simulink library "AFCToolbox2023a"  (R2023a)
settings: Solver=VariableStepAuto  StartTime=0.0  StopTime=10.0  RelTol=1e-3
undefined symbols (not defined in the file or in its folder): AFC5Toolbox_SimuMoudle, AFCToolbox, ax, ay, az, btnSample, C_d, C_dm, C_m, C_t, Control, d, declination_table, dp0, dp1, dp2, dp3, dt, euler_0, g0, I_xyz, inclination_table, J_m, lmd_high, lmd_low, lp_acc_knoise, lp_acc_max, lp_acc_min, lp_acc_seed, lp_GPS_BL_max, lp_GPS_BL_min, lp_GPS_H_max, lp_GPS_H_min, lp_GPS_knoise, lp_GPS_seed, lp_GPS_vel_max, lp_GPS_vel_min, lp_gyro_knoise, lp_gyro_max, lp_gyro_min, lp_gyro_seed, lp_hf_vwind, lp_hs_vwind_interp, lp_kaerorho, lp_kaeroT, lp_kIxyz, lp_kmass, lp_momentx_A0, lp_momentx_Af, lp_momentx_ts, lp_momenty_A0, lp_momenty_Af, lp_momenty_ts, lp_momentz_A0, lp_momentz_Af, lp_momentz_ts, lp_vf_vwind, lp_vs_vwind_interp, lp_vwind_thetax, lp_vwind_thetaz ... (+54)
libraries: $bdroot x104, simulink x75, etargetslib x32, sharedtransform x13, simulink_extras x12, dspstat3 x11, aerolibconvert2 x9, aerolibtransform2 x3, aerolibutil x2, matrix_library x1
(part 9 of 10)

== matlab function AFCToolbox2023a/基础导航算法模型库/ECL EKF/Subsystem/Subsystem2/Predict Covariance ==
  data: delta_ang input; delta_vel input; P output; states input; P input single; dt input; accel_bias_inhibit input
function P  = PredictCovariance(delta_ang, ...%imu_sample_delayed.delta_ang
    delta_vel,...%imu_sample_delayed.delta_vel
    states,...% previous state vector (4x1 quaternion, 3x1 velocity, 3x1 position, 3x1 delAng bias, 3x1 delVel bias)
    P, dt, ... % IMU and prediction time step
    accel_bias_inhibit)% inhibited for the specified axis
    

%  the current status of the filter control modes
%% control status flags
control_status_flags.wind  = 1;
control_status_flags.mag_3D = 1;

% tuning parameters
%% InitCovariance params
params.gps_vel_noise = 0.5;
params.gps_pos_noise = 0.5;
params.pos_noaid_noise = 10;
params.baro_noise = 2;
params.switch_on_gyro_bias = 0.1;
params.switch_on_accel_bias = 0.2;
params.mag_noise = 0.05;
params.initial_wind_uncertainty = 1;
params.gyro_noise = 0.00001;
params.accel_noise = 0.35;
%% PredictCovariance params
params.gyro_bias_p_noise = 0.0001;
params.accel_bias_p_noise = 0.001;
params.mage_p_noise = 0.001;
params.magb_p_noise = 0.0001;
params.wind_vel_p_noise = 0.5;


%% assign intermediate state variables
% quaternion
states_quat_nominal = normQuat(states(1:4));
q0 = states_quat_nominal(1);
q1 = states_quat_nominal(2);
q2 = states_quat_nominal(3);
q3 = states_quat_nominal(4);
% delta angle 
dax = delta_ang(1);
day = delta_ang(2);
daz = delta_ang(3);
% delta velocity
dvx = delta_vel(1);
dvy = delta_vel(2);
dvz = delta_vel(3);
% delta angle bias
dax_b = states(11);
day_b = states(12);
daz_b = states(13);
% delta velocity bias
dvx_b = states(14);
dvy_b = states(15);
dvz_b = states(16);

% convert rate of change of rate gyro bias (rad/s**2) as specified by the parameter to an expected change in delta angle (rad) since the last update
d_ang_bias_sig = dt * dt * params.gyro_bias_p_noise;

% convert rate of change of accelerometer bias (m/s**3) as specified by the parameter to an expected change in delta velocity (m/s) since the last update
d_vel_bias_sig = dt * dt * params.accel_bias_p_noise;

%% This process noise determines the rate of estimation of IMU bias errors
% Set filter state process noise other than IMU errors, which are already
% built into the derived covariance prediction equations.
mag_I_sig = dt * params.mage_p_noise;
mag_B_sig = dt * params.magb_p_noise;
wind_vel_sig = dt * params.wind_vel_p_noise;
process_noise = [zeros(1,10), d_ang_bias_sig*[1 1 1], d_vel_bias_sig*[1 1 1], mag_I_sig*[1 1 1], mag_B_sig*[1 1 1], wind_vel_sig*[1 1]].^2;

%% assign IMU noise variances
% Specify the noise variance on the IMU delta angles and delta velocities
daxVar = (dt * params.gyro_noise)^2;
dayVar = daxVar;
dazVar = daxVar;
dvxVar = (dt * params.accel_noise)^2;
dvyVar = dvxVar;
dvzVar = dvxVar;

%% intermediate calculations——求解223条赋值语句，得出中间变量
PS0 = power(q1, 2);
PS1 = 0.25*daxVar;
PS2 = power(q2, 2);
PS3 = 0.25*dayVar;
PS4 = power(q3, 2);
PS5 = 0.25*dazVar;
PS6 = 0.5*q1;
PS7 = 0.5*q2;
PS8 = C_P(P,10,11)*PS7;
PS9 = 0.5*q3;
PS10 = C_P(P,10,12)*PS9;
PS11 = 0.5*dax - 0.5*dax_b;
PS12 = 0.5*day - 0.5*day_b;
PS13 = 0.5*daz - 0.5*daz_b;
PS14 = C_P(P,0,10) - C_P(P,1,10)*PS11 + C_P(P,10,10)*PS6 - C_P(P,2,10)*PS12 - C_P(P,3,10)*PS13 + PS10 + PS8;
PS15 = C_P(P,10,11)*PS6;
PS16 = C_P(P,11,12)*PS9;
PS17 = C_P(P,0,11) - C_P(P,1,11)*PS11 + C_P(P,11,11)*PS7 - C_P(P,2,11)*PS12 - C_P(P,3,11)*PS13 + PS15 + PS16;
PS18 = C_P(P,10,12)*PS6;
PS19 = C_P(P,11,12)*PS7;
PS20 = C_P(P,0,12) - C_P(P,1,12)*PS11 + C_P(P,12,12)*PS9 - C_P(P,2,12)*PS12 - C_P(P,3,12)*PS13 + PS18 + PS19;
PS21 = C_P(P,1,2)*PS12;
PS22 = -C_P(P,1,3)*PS13;
PS23 = C_P(P,0,1) - C_P(P,1,1)*PS11 + C_P(P,1,10)*PS6 + C_P(P,1,11)*PS7 + C_P(P,1,12)*PS9 - PS21 + PS22;
PS24 = -C_P(P,1,2)*PS11;
PS25 = C_P(P,2,3)*PS13;
PS26 = C_P(P,0,2) + C_P(P,2,10)*PS6 + C_P(P,2,11)*PS7 + C_P(P,2,12)*PS9 - C_P(P,2,2)*PS12 + PS24 - PS25;
PS27 = C_P(P,1,3)*PS11;
PS28 = -C_P(P,2,3)*PS12;
PS29 = C_P(P,0,3) + C_P(P,3,10)*PS6 + C_P(P,3,11)*PS7 + C_P(P,3,12)*PS9 - C_P(P,3,3)*PS13 - PS27 + PS28;
PS30 = C_P(P,0,1)*PS11;
PS31 = C_P(P,0,2)*PS12;
PS32 = C_P(P,0,3)*PS13;
PS33 = C_P(P,0,0) + C_P(P,0,10)*PS6 + C_P(P,0,11)*PS7 + C_P(P,0,12)*PS9 - PS30 - PS31 - PS32;
PS34 = 0.5*q0;
PS35 = q2*q3;
PS36 = q0*q1;
PS37 = q1*q3;
PS38 = q0*q2;
PS39 = q1*q2;
PS40 = q0*q3;
PS41 = 2*PS2;
PS42 = 2*PS4 - 1;
PS43 = PS41 + PS42;
PS44 = C_P(P,0,13) - C_P(P,1,13)*PS11 + C_P(P,10,13)*PS6 + C_P(P,11,13)*PS7 + C_P(P,12,13)*PS9 - C_P(P,2,13)*PS12 - C_P(P,3,13)*PS13;
PS45 = PS37 + PS38;
PS46 = C_P(P,0,15) - C_P(P,1,15)*PS11 + C_P(P,10,15)*PS6 + C_P(P,11,15)*PS7 + C_P(P,12,15)*PS9 - C_P(P,2,15)*PS12 - C_P(P,3,15)*PS13;
PS47 = 2*PS46;
PS48 = dvy - dvy_b;
PS49 = PS48*q0;
PS50 = dvz - dvz_b;
PS51 = PS50*q1;
PS52 = dvx - dvx_b;
PS53 = PS52*q3;
PS54 = PS49 - PS51 + 2*PS53;
PS55 = 2*PS29;
PS56 = -PS39 + PS40;
PS57 = C_P(P,0,14) - C_P(P,1,14)*PS11 + C_P(P,10,14)*PS6 + C_P(P,11,14)*PS7 + C_P(P,12,14)*PS9 - C_P(P,2,14)*PS12 - C_P(P,3,14)*PS13;
PS58 = 2*PS57;
PS59 = PS48*q2;
PS60 = PS50*q3;
PS61 = PS59 + PS60;
PS62 = 2*PS23;
PS63 = PS50*q2;
PS64 = PS48*q3;
PS65 = -PS64;
PS66 = PS63 + PS65;
PS67 = 2*PS33;
PS68 = PS50*q0;
PS69 = PS48*q1;
PS70 = PS52*q2;
PS71 = PS68 + PS69 - 2*PS70;
PS72 = 2*PS26;
PS73 = C_P(P,0,4) - C_P(P,1,4)*PS11 - C_P(P,2,4)*PS12 - C_P(P,3,4)*PS13 + C_P(P,4,10)*PS6 + C_P(P,4,11)*PS7 + C_P(P,4,12)*PS9;
PS74 = 2*PS0;
PS75 = PS42 + PS74;
PS76 = PS39 + PS40;
PS77 = 2*PS44;
PS78 = PS51 - PS53;
PS79 = -PS70;
PS80 = PS68 + 2*PS69 + PS79;
PS81 = -PS35 + PS36;
PS82 = PS52*q1;
PS83 = PS60 + PS82;
PS84 = PS52*q0;
PS85 = PS63 - 2*PS64 + PS84;
PS86 = C_P(P,0,5) - C_P(P,1,5)*PS11 - C_P(P,2,5)*PS12 - C_P(P,3,5)*PS13 + C_P(P,5,10)*PS6 + C_P(P,5,11)*PS7 + C_P(P,5,12)*PS9;
PS87 = PS41 + PS74 - 1;
PS88 = PS35 + PS36;
PS89 = 2*PS63 + PS65 + PS84;
PS90 = -PS37 + PS38;
PS91 = PS59 + PS82;
PS92 = PS69 + PS79;
PS93 = PS49 - 2*PS51 + PS53;
PS94 = C_P(P,0,6) - C_P(P,1,6)*PS11 - C_P(P,2,6)*PS12 - C_P(P,3,6)*PS13 + C_P(P,6,10)*PS6 + C_P(P,6,11)*PS7 + C_P(P,6,12)*PS9;
PS95 = power(q0, 2);
PS96 = -C_P(P,10,11)*PS34;
PS97 = C_P(P,0,11)*PS11 + C_P(P,1,11) + C_P(P,11,11)*PS9 + C_P(P,2,11)*PS13 - C_P(P,3,11)*PS12 - PS19 + PS96;
PS98 = C_P(P,0,2)*PS13;
PS99 = C_P(P,0,3)*PS12;
PS100 = C_P(P,0,0)*PS11 + C_P(P,0,1) - C_P(P,0,10)*PS34 + C_P(P,0,11)*PS9 - C_P(P,0,12)*PS7 + PS98 - PS99;
PS101 = C_P(P,0,2)*PS11;
PS102 = C_P(P,1,2) - C_P(P,2,10)*PS34 + C_P(P,2,11)*PS9 - C_P(P,2,12)*PS7 + C_P(P,2,2)*PS13 + PS101 + PS28;
PS103 = C_P(P,10,11)*PS9;
PS104 = C_P(P,10,12)*PS7;
PS105 = C_P(P,0,10)*PS11 + C_P(P,1,10) - C_P(P,10,10)*PS34 + C_P(P,2,10)*PS13 - C_P(P,3,10)*PS12 + PS103 - PS104;
PS106 = -C_P(P,10,12)*PS34;
PS107 = C_P(P,0,12)*PS11 + C_P(P,1,12) - C_P(P,12,12)*PS7 + C_P(P,2,12)*PS13 - C_P(P,3,12)*PS12 + PS106 + PS16;
PS108 = C_P(P,0,3)*PS11;
PS109 = C_P(P,1,3) - C_P(P,3,10)*PS34 + C_P(P,3,11)*PS9 - C_P(P,3,12)*PS7 - C_P(P,3,3)*PS12 + PS108 + PS25;
PS110 = C_P(P,1,2)*PS13;
PS111 = C_P(P,1,3)*PS12;
PS112 = C_P(P,1,1) - C_P(P,1,10)*PS34 + C_P(P,1,11)*PS9 - C_P(P,1,12)*PS7 + PS110 - PS111 + PS30;
PS113 = C_P(P,0,13)*PS11 + C_P(P,1,13) - C_P(P,10,13)*PS34 + C_P(P,11,13)*PS9 - C_P(P,12,13)*PS7 + C_P(P,2,13)*PS13 - C_P(P,3,13)*PS12;
PS114 = C_P(P,0,15)*PS11 + C_P(P,1,15) - C_P(P,10,15)*PS34 + C_P(P,11,15)*PS9 - C_P(P,12,15)*PS7 + C_P(P,2,15)*PS13 - C_P(P,3,15)*PS12;
PS115 = 2*PS114;
PS116 = 2*PS109;
PS117 = C_P(P,0,14)*PS11 + C_P(P,1,14) - C_P(P,10,14)*PS34 + C_P(P,11,14)*PS9 - C_P(P,12,14)*PS7 + C_P(P,2,14)*PS13 - C_P(P,3,14)*PS12;
PS118 = 2*PS117;
PS119 = 2*PS112;
PS120 = 2*PS100;
PS121 = 2*PS102;
PS122 = C_P(P,0,4)*PS11 + C_P(P,1,4) + C_P(P,2,4)*PS13 - C_P(P,3,4)*PS12 - C_P(P,4,10)*PS34 + C_P(P,4,11)*PS9 - C_P(P,4,12)*PS7;
PS123 = 2*PS113;
PS124 = C_P(P,0,5)*PS11 + C_P(P,1,5) + C_P(P,2,5)*PS13 - C_P(P,3,5)*PS12 - C_P(P,5,10)*PS34 + C_P(P,5,11)*PS9 - C_P(P,5,12)*PS7;
PS125 = C_P(P,0,6)*PS11 + C_P(P,1,6) + C_P(P,2,6)*PS13 - C_P(P,3,6)*PS12 - C_P(P,6,10)*PS34 + C_P(P,6,11)*PS9 - C_P(P,6,12)*PS7;
PS126 = -C_P(P,11,12)*PS34;
PS127 = C_P(P,0,12)*PS12 - C_P(P,1,12)*PS13 + C_P(P,12,12)*PS6 + C_P(P,2,12) + C_P(P,3,12)*PS11 - PS10 + PS126;
PS128 = C_P(P,2,3) - C_P(P,3,10)*PS9 - C_P(P,3,11)*PS34 + C_P(P,3,12)*PS6 + C_P(P,3,3)*PS11 + PS22 + PS99;
PS129 = C_P(P,0,1)*PS13;
PS130 = C_P(P,0,0)*PS12 - C_P(P,0,10)*PS9 - C_P(P,0,11)*PS34 + C_P(P,0,12)*PS6 + C_P(P,0,2) + PS108 - PS129;
PS131 = C_P(P,11,12)*PS6;
PS132 = C_P(P,0,11)*PS12 - C_P(P,1,11)*PS13 - C_P(P,11,11)*PS34 + C_P(P,2,11) + C_P(P,3,11)*PS11 - PS103 + PS131;
PS133 = C_P(P,0,10)*PS12 - C_P(P,1,10)*PS13 - C_P(P,10,10)*PS9 + C_P(P,2,10) + C_P(P,3,10)*PS11 + PS18 + PS96;
PS134 = C_P(P,0,1)*PS12;
PS135 = -C_P(P,1,1)*PS13 - C_P(P,1,10)*PS9 - C_P(P,1,11)*PS34 + C_P(P,1,12)*PS6 + C_P(P,1,2) + PS134 + PS27;
PS136 = C_P(P,2,3)*PS11;
PS137 = -C_P(P,2,10)*PS9 - C_P(P,2,11)*PS34 + C_P(P,2,12)*PS6 + C_P(P,2,2) - PS110 + PS136 + PS31;
PS138 = C_P(P,0,13)*PS12 - C_P(P,1,13)*PS13 - C_P(P,10,13)*PS9 - C_P(P,11,13)*PS34 + C_P(P,12,13)*PS6 + C_P(P,2,13) + C_P(P,3,13)*PS11;
PS139 = C_P(P,0,15)*PS12 - C_P(P,1,15)*PS13 - C_P(P,10,15)*PS9 - C_P(P,11,15)*PS34 + C_P(P,12,15)*PS6 + C_P(P,2,15) + C_P(P,3,15)*PS11;
PS140 = 2*PS139;
PS141 = 2*PS128;
PS142 = C_P(P,0,14)*PS12 - C_P(P,1,14)*PS13 - C_P(P,10,14)*PS9 - C_P(P,11,14)*PS34 + C_P(P,12,14)*PS6 + C_P(P,2,14) + C_P(P,3,14)*PS11;
PS143 = 2*PS142;
PS144 = 2*PS135;
PS145 = 2*PS130;
PS146 = 2*PS137;
PS147 = C_P(P,0,4)*PS12 - C_P(P,1,4)*PS13 + C_P(P,2,4) + C_P(P,3,4)*PS11 - C_P(P,4,10)*PS9 - C_P(P,4,11)*PS34 + C_P(P,4,12)*PS6;
PS148 = 2*PS138;
PS149 = C_P(P,0,5)*PS12 - C_P(P,1,5)*PS13 + C_P(P,2,5) + C_P(P,3,5)*PS11 - C_P(P,5,10)*PS9 - C_P(P,5,11)*PS34 + C_P(P,5,12)*PS6;
PS150 = C_P(P,0,6)*PS12 - C_P(P,1,6)*PS13 + C_P(P,2,6) + C_P(P,3,6)*PS11 - C_P(P,6,10)*PS9 - C_P(P,6,11)*PS34 + C_P(P,6,12)*PS6;
PS151 = C_P(P,0,10)*PS13 + C_P(P,1,10)*PS12 + C_P(P,10,10)*PS7 - C_P(P,2,10)*PS11 + C_P(P,3,10) + PS106 - PS15;
PS152 = C_P(P,1,1)*PS12 + C_P(P,1,10)*PS7 - C_P(P,1,11)*PS6 - C_P(P,1,12)*PS34 + C_P(P,1,3) + PS129 + PS24;
PS153 = C_P(P,0,0)*PS13 + C_P(P,0,10)*PS7 - C_P(P,0,11)*PS6 - C_P(P,0,12)*PS34 + C_P(P,0,3) - PS101 + PS134;
PS154 = C_P(P,0,12)*PS13 + C_P(P,1,12)*PS12 - C_P(P,12,12)*PS34 - C_P(P,2,12)*PS11 + C_P(P,3,12) + PS104 - PS131;
PS155 = C_P(P,0,11)*PS13 + C_P(P,1,11)*PS12 - C_P(P,11,11)*PS6 - C_P(P,2,11)*PS11 + C_P(P,3,11) + PS126 + PS8;
PS156 = C_P(P,2,10)*PS7 - C_P(P,2,11)*PS6 - C_P(P,2,12)*PS34 - C_P(P,2,2)*PS11 + C_P(P,2,3) + PS21 + PS98;
PS157 = C_P(P,3,10)*PS7 - C_P(P,3,11)*PS6 - C_P(P,3,12)*PS34 + C_P(P,3,3) + PS111 - PS136 + PS32;
PS158 = C_P(P,0,13)*PS13 + C_P(P,1,13)*PS12 + C_P(P,10,13)*PS7 - C_P(P,11,13)*PS6 - C_P(P,12,13)*PS34 - C_P(P,2,13)*PS11 + C_P(P,3,13);
PS159 = C_P(P,0,15)*PS13 + C_P(P,1,15)*PS12 + C_P(P,10,15)*PS7 - C_P(P,11,15)*PS6 - C_P(P,12,15)*PS34 - C_P(P,2,15)*PS11 + C_P(P,3,15);
PS160 = 2*PS159;
PS161 = 2*PS157;
PS162 = C_P(P,0,14)*PS13 + C_P(P,1,14)*PS12 + C_P(P,10,14)*PS7 - C_P(P,11,14)*PS6 - C_P(P,12,14)*PS34 - C_P(P,2,14)*PS11 + C_P(P,3,14);
PS163 = 2*PS162;
PS164 = 2*PS152;
PS165 = 2*PS153;
PS166 = 2*PS156;
PS167 = C_P(P,0,4)*PS13 + C_P(P,1,4)*PS12 - C_P(P,2,4)*PS11 + C_P(P,3,4) + C_P(P,4,10)*PS7 - C_P(P,4,11)*PS6 - C_P(P,4,12)*PS34;
PS168 = 2*PS158;
PS169 = C_P(P,0,5)*PS13 + C_P(P,1,5)*PS12 - C_P(P,2,5)*PS11 + C_P(P,3,5) + C_P(P,5,10)*PS7 - C_P(P,5,11)*PS6 - C_P(P,5,12)*PS34;
PS170 = C_P(P,0,6)*PS13 + C_P(P,1,6)*PS12 - C_P(P,2,6)*PS11 + C_P(P,3,6) + C_P(P,6,10)*PS7 - C_P(P,6,11)*PS6 - C_P(P,6,12)*PS34;
PS171 = 2*PS45;
PS172 = 2*PS56;
PS173 = 2*PS61;
PS174 = 2*PS66;
PS175 = 2*PS71;
PS176 = 2*PS54;
PS177 = C_P(P,0,13)*PS174 + C_P(P,1,13)*PS173 + C_P(P,13,13)*PS43 + C_P(P,13,14)*PS172 - C_P(P,13,15)*PS171 + C_P(P,2,13)*PS175 - C_P(P,3,13)*PS176 + C_P(P,4,13);
PS178 = C_P(P,0,15)*PS174 + C_P(P,1,15)*PS173 + C_P(P,13,15)*PS43 + C_P(P,14,15)*PS172 - C_P(P,15,15)*PS171 + C_P(P,2,15)*PS175 - C_P(P,3,15)*PS176 + C_P(P,4,15);
PS179 = C_P(P,0,3)*PS174 + C_P(P,1,3)*PS173 + C_P(P,2,3)*PS175 + C_P(P,3,13)*PS43 + C_P(P,3,14)*PS172 - C_P(P,3,15)*PS171 - C_P(P,3,3)*PS176 + C_P(P,3,4);
PS180 = C_P(P,0,14)*PS174 + C_P(P,1,14)*PS173 + C_P(P,13,14)*PS43 + C_P(P,14,14)*PS172 - C_P(P,14,15)*PS171 + C_P(P,2,14)*PS175 - C_P(P,3,14)*PS176 + C_P(P,4,14);
PS181 = C_P(P,0,1)*PS174 + C_P(P,1,1)*PS173 + C_P(P,1,13)*PS43 + C_P(P,1,14)*PS172 - C_P(P,1,15)*PS171 + C_P(P,1,2)*PS175 - C_P(P,1,3)*PS176 + C_P(P,1,4);
PS182 = C_P(P,0,0)*PS174 + C_P(P,0,1)*PS173 + C_P(P,0,13)*PS43 + C_P(P,0,14)*PS172 - C_P(P,0,15)*PS171 + C_P(P,0,2)*PS175 - C_P(P,0,3)*PS176 + C_P(P,0,4);
PS183 = C_P(P,0,2)*PS174 + C_P(P,1,2)*PS173 + C_P(P,2,13)*PS43 + C_P(P,2,14)*PS172 - C_P(P,2,15)*PS171 + C_P(P,2,2)*PS175 - C_P(P,2,3)*PS176 + C_P(P,2,4);
PS184 = 4*dvyVar;
PS185 = 4*dvzVar;
PS186 = C_P(P,0,4)*PS174 + C_P(P,1,4)*PS173 + C_P(P,2,4)*PS175 - C_P(P,3,4)*PS176 + C_P(P,4,13)*PS43 + C_P(P,4,14)*PS172 - C_P(P,4,15)*PS171 + C_P(P,4,4);
PS187 = 2*PS177;
PS188 = 2*PS182;
PS189 = 2*PS181;
PS190 = 2*PS81;
PS191 = 2*PS183;
PS192 = 2*PS179;
PS193 = 2*PS76;
PS194 = PS43*dvxVar;
PS195 = PS75*dvyVar;
PS196 = C_P(P,0,5)*PS174 + C_P(P,1,5)*PS173 + C_P(P,2,5)*PS175 - C_P(P,3,5)*PS176 + C_P(P,4,5) + C_P(P,5,13)*PS43 + C_P(P,5,14)*PS172 - C_P(P,5,15)*PS171;
PS197 = 2*PS88;
PS198 = PS87*dvzVar;
PS199 = 2*PS90;
PS200 = C_P(P,0,6)*PS174 + C_P(P,1,6)*PS173 + C_P(P,2,6)*PS175 - C_P(P,3,6)*PS176 + C_P(P,4,6) + C_P(P,6,13)*PS43 + C_P(P,6,14)*PS172 - C_P(P,6,15)*PS171;
PS201 = 2*PS83;
PS202 = 2*PS78;
PS203 = 2*PS85;
PS204 = 2*PS80;
PS205 = -C_P(P,0,14)*PS202 - C_P(P,1,14)*PS204 - C_P(P,13,14)*PS193 + C_P(P,14,14)*PS75 + C_P(P,14,15)*PS190 + C_P(P,2,14)*PS201 + C_P(P,3,14)*PS203 + C_P(P,5,14);
PS206 = -C_P(P,0,13)*PS202 - C_P(P,1,13)*PS204 - C_P(P,13,13)*PS193 + C_P(P,13,14)*PS75 + C_P(P,13,15)*PS190 + C_P(P,2,13)*PS201 + C_P(P,3,13)*PS203 + C_P(P,5,13);
PS207 = -C_P(P,0,0)*PS202 - C_P(P,0,1)*PS204 - C_P(P,0,13)*PS193 + C_P(P,0,14)*PS75 + C_P(P,0,15)*PS190 + C_P(P,0,2)*PS201 + C_P(P,0,3)*PS203 + C_P(P,0,5);
PS208 = -C_P(P,0,1)*PS202 - C_P(P,1,1)*PS204 - C_P(P,1,13)*PS193 + C_P(P,1,14)*PS75 + C_P(P,1,15)*PS190 + C_P(P,1,2)*PS201 + C_P(P,1,3)*PS203 + C_P(P,1,5);
PS209 = -C_P(P,0,15)*PS202 - C_P(P,1,15)*PS204 - C_P(P,13,15)*PS193 + C_P(P,14,15)*PS75 + C_P(P,15,15)*PS190 + C_P(P,2,15)*PS201 + C_P(P,3,15)*PS203 + C_P(P,5,15);
PS210 = -C_P(P,0,2)*PS202 - C_P(P,1,2)*PS204 - C_P(P,2,13)*PS193 + C_P(P,2,14)*PS75 + C_P(P,2,15)*PS190 + C_P(P,2,2)*PS201 + C_P(P,2,3)*PS203 + C_P(P,2,5);
PS211 = -C_P(P,0,3)*PS202 - C_P(P,1,3)*PS204 + C_P(P,2,3)*PS201 - C_P(P,3,13)*PS193 + C_P(P,3,14)*PS75 + C_P(P,3,15)*PS190 + C_P(P,3,3)*PS203 + C_P(P,3,5);
PS212 = 4*dvxVar;
PS213 = -C_P(P,0,5)*PS202 - C_P(P,1,5)*PS204 + C_P(P,2,5)*PS201 + C_P(P,3,5)*PS203 - C_P(P,5,13)*PS193 + C_P(P,5,14)*PS75 + C_P(P,5,15)*PS190 + C_P(P,5,5);
PS214 = 2*PS89;
PS215 = 2*PS91;
PS216 = 2*PS92;
PS217 = 2*PS93;
PS218 = -C_P(P,0,6)*PS202 - C_P(P,1,6)*PS204 + C_P(P,2,6)*PS201 + C_P(P,3,6)*PS203 + C_P(P,5,6) - C_P(P,6,13)*PS193 + C_P(P,6,14)*PS75 + C_P(P,6,15)*PS190;
PS219 = C_P(P,0,15)*PS216 + C_P(P,1,15)*PS217 + C_P(P,13,15)*PS199 - C_P(P,14,15)*PS197 + C_P(P,15,15)*PS87 - C_P(P,2,15)*PS214 + C_P(P,3,15)*PS215 + C_P(P,6,15);
PS220 = C_P(P,0,14)*PS216 + C_P(P,1,14)*PS217 + C_P(P,13,14)*PS199 - C_P(P,14,14)*PS197 + C_P(P,14,15)*PS87 - C_P(P,2,14)*PS214 + C_P(P,3,14)*PS215 + C_P(P,6,14);
PS221 = C_P(P,0,13)*PS216 + C_P(P,1,13)*PS217 + C_P(P,13,13)*PS199 - C_P(P,13,14)*PS197 + C_P(P,13,15)*PS87 - C_P(P,2,13)*PS214 + C_P(P,3,13)*PS215 + C_P(P,6,13);
PS222 = C_P(P,0,6)*PS216 + C_P(P,1,6)*PS217 - C_P(P,2,6)*PS214 + C_P(P,3,6)*PS215 + C_P(P,6,13)*PS199 - C_P(P,6,14)*PS197 + C_P(P,6,15)*PS87 + C_P(P,6,6);

%% caculate covariances
% initialize covariances
nextP_ = zeros(24,24);
% calculate variances and upper diagonal covariances for QUATERNION, VELOCITY, POSITION AND GYRO BIAS states
nextP_(1,1) = PS0*PS1 - PS11*PS23 - PS12*PS26 - PS13*PS29 + PS14*PS6 + PS17*PS7 + PS2*PS3 + PS20*PS9 + PS33 + PS4*PS5;
nextP_(1,2) = -PS1*PS36 + PS11*PS33 - PS12*PS29 + PS13*PS26 - PS14*PS34 + PS17*PS9 - PS20*PS7 + PS23 + PS3*PS35 - PS35*PS5;
nextP_(2,2) = PS1*PS95 + PS100*PS11 + PS102*PS13 - PS105*PS34 - PS107*PS7 - PS109*PS12 + PS112 + PS2*PS5 + PS3*PS4 + PS9*PS97;

nextP_(1,3) = -PS1*PS37 + PS11*PS29 + PS12*PS33 - PS13*PS23 - PS14*PS9 - PS17*PS34 + PS20*PS6 + PS26 - PS3*PS38 + PS37*PS5;
nextP_(2,3) = PS1*PS40 + PS100*PS12 + PS102 - PS105*PS9 + PS107*PS6 + PS109*PS11 - PS112*PS13 - PS3*PS40 - PS34*PS97 - PS39*PS5;
nextP_(3,3) = PS0*PS5 + PS1*PS4 + PS11*PS128 + PS12*PS130 + PS127*PS6 - PS13*PS135 - PS132*PS34 - PS133*PS9 + PS137 + PS3*PS95;

nextP_(1,4) = PS1*PS39 - PS11*PS26 + PS12*PS23 + PS13*PS33 + PS14*PS7 - PS17*PS6 - PS20*PS34 + PS29 - PS3*PS39 - PS40*PS5;
nextP_(2,4) = -PS1*PS38 + PS100*PS13 - PS102*PS11 + PS105*PS7 - PS107*PS34 + PS109 + PS112*PS12 - PS3*PS37 + PS38*PS5 - PS6*PS97;
nextP_(3,4) = -PS1*PS35 - PS11*PS137 + PS12*PS135 - PS127*PS34 + PS128 + PS13*PS130 - PS132*PS6 + PS133*PS7 + PS3*PS36 - PS36*PS5;
nextP_(4,4) = PS0*PS3 + PS1*PS2 - PS11*PS156 + PS12*PS152 + PS13*PS153 + PS151*PS7 - PS154*PS34 - PS155*PS6 + PS157 + PS5*PS95;

nextP_(1,5) = PS43*PS44 - PS45*PS47 - PS54*PS55 + PS56*PS58 + PS61*PS62 + PS66*PS67 + PS71*PS72 + PS73;
nextP_(2,5) = PS113*PS43 - PS115*PS45 - PS116*PS54 + PS118*PS56 + PS119*PS61 + PS120*PS66 + PS121*PS71 + PS122;
nextP_(3,5) = PS138*PS43 - PS140*PS45 - PS141*PS54 + PS143*PS56 + PS144*PS61 + PS145*PS66 + PS146*PS71 + PS147;
nextP_(4,5) = PS158*PS43 - PS160*PS45 - PS161*PS54 + PS163*PS56 + PS164*PS61 + PS165*PS66 + PS166*PS71 + PS167;
nextP_(5,5) = -PS171*PS178 + PS172*PS180 + PS173*PS181 + PS174*PS182 + PS175*PS183 - PS176*PS179 + PS177*PS43 + PS184*power(PS56, 2) + PS185*power(PS45, 2) + PS186 + power(PS43, 2)*dvxVar;

nextP_(1,6) = PS47*PS81 + PS55*PS85 + PS57*PS75 - PS62*PS80 - PS67*PS78 + PS72*PS83 - PS76*PS77 + PS86;
nextP_(2,6) = PS115*PS81 + PS116*PS85 + PS117*PS75 - PS119*PS80 - PS120*PS78 + PS121*PS83 - PS123*PS76 + PS124;
nextP_(3,6) = PS140*PS81 + PS141*PS85 + PS142*PS75 - PS144*PS80 - PS145*PS78 + PS146*PS83 - PS148*PS76 + PS149;
nextP_(4,6) = PS160*PS81 + PS161*PS85 + PS162*PS75 - PS164*PS80 - PS165*PS78 + PS166*PS83 - PS168*PS76 + PS169;
nextP_(5,6) = PS172*PS195 + PS178*PS190 + PS180*PS75 - PS185*PS45*PS81 - PS187*PS76 - PS188*PS78 - PS189*PS80 + PS191*PS83 + PS192*PS85 - PS193*PS194 + PS196;
nextP_(6,6) = PS185*power(PS81, 2) + PS190*PS209 - PS193*PS206 + PS201*PS210 - PS202*PS207 + PS203*PS211 - PS204*PS208 + PS205*PS75 + PS212*power(PS76, 2) + PS213 + power(PS75, 2)*dvyVar;

nextP_(1,7) = PS46*PS87 + PS55*PS91 - PS58*PS88 + PS62*PS93 + PS67*PS92 - PS72*PS89 + PS77*PS90 + PS94;
nextP_(2,7) = PS114*PS87 + PS116*PS91 - PS118*PS88 + PS119*PS93 + PS120*PS92 - PS121*PS89 + PS123*PS90 + PS125;
nextP_(3,7) = PS139*PS87 + PS141*PS91 - PS143*PS88 + PS144*PS93 + PS145*PS92 - PS146*PS89 + PS148*PS90 + PS150;
nextP_(4,7) = PS159*PS87 + PS161*PS91 - PS163*PS88 + PS164*PS93 + PS165*PS92 - PS166*PS89 + PS168*PS90 + PS170;
nextP_(5,7) = -PS171*PS198 + PS178*PS87 - PS180*PS197 - PS184*PS56*PS88 + PS187*PS90 + PS188*PS92 + PS189*PS93 - PS191*PS89 + PS192*PS91 + PS194*PS199 + PS200;
nextP_(6,7) = PS190*PS198 - PS195*PS197 - PS197*PS205 + PS199*PS206 + PS207*PS216 + PS208*PS217 + PS209*PS87 - PS210*PS214 + PS211*PS215 - PS212*PS76*PS90 + PS218;
nextP_(7,7) = PS184*power(PS88, 2) - PS197*PS220 + PS199*PS221 + PS212*power(PS90, 2) - PS214*(C_P(P,0,2)*PS216 + C_P(P,1,2)*PS217 + C_P(P,2,13)*PS199 - C_P(P,2,14)*PS197 + C_P(P,2,15)*PS87 - C_P(P,2,2)*PS214 + C_P(P,2,3)*PS215 + C_P(P,2,6)) + PS215*(C_P(P,0,3)*PS216 + C_P(P,1,3)*PS217 - C_P(P,2,3)*PS214 + C_P(P,3,13)*PS199 - C_P(P,3,14)*PS197 + C_P(P,3,15)*PS87 + C_P(P,3,3)*PS215 + C_P(P,3,6)) + PS216*(C_P(P,0,0)*PS216 + C_P(P,0,1)*PS217 + C_P(P,0,13)*PS199 - C_P(P,0,14)*PS197 + C_P(P,0,15)*PS87 - C_P(P,0,2)*PS214 + C_P(P,0,3)*PS215 + C_P(P,0,6)) + PS217*(C_P(P,0,1)*PS216 + C_P(P,1,1)*PS217 + C_P(P,1,13)*PS199 - C_P(P,1,14)*PS197 + C_P(P,1,15)*PS87 - C_P(P,1,2)*PS214 + C_P(P,1,3)*PS215 + C_P(P,1,6)) + PS219*PS87 + PS222 + power(PS87, 2)*dvzVar;

nextP_(1,8) = C_P(P,0,7) - C_P(P,1,7)*PS11 - C_P(P,2,7)*PS12 - C_P(P,3,7)*PS13 + C_P(P,7,10)*PS6 + C_P(P,7,11)*PS7 + C_P(P,7,12)*PS9 + PS73*dt;
nextP_(2,8) = C_P(P,0,7)*PS11 + C_P(P,1,7) + C_P(P,2,7)*PS13 - C_P(P,3,7)*PS12 - C_P(P,7,10)*PS34 + C_P(P,7,11)*PS9 - C_P(P,7,12)*PS7 + PS122*dt;
nextP_(3,8) = C_P(P,0,7)*PS12 - C_P(P,1,7)*PS13 + C_P(P,2,7) + C_P(P,3,7)*PS11 - C_P(P,7,10)*PS9 - C_P(P,7,11)*PS34 + C_P(P,7,12)*PS6 + PS147*dt;
nextP_(4,8) = C_P(P,0,7)*PS13 + C_P(P,1,7)*PS12 - C_P(P,2,7)*PS11 + C_P(P,3,7) + C_P(P,7,10)*PS7 - C_P(P,7,11)*PS6 - C_P(P,7,12)*PS34 + PS167*dt;
nextP_(5,8) = C_P(P,0,7)*PS174 + C_P(P,1,7)*PS173 + C_P(P,2,7)*PS175 - C_P(P,3,7)*PS176 + C_P(P,4,7) + C_P(P,7,13)*PS43 + C_P(P,7,14)*PS172 - C_P(P,7,15)*PS171 + PS186*dt;
nextP_(6,8) = -C_P(P,0,7)*PS202 - C_P(P,1,7)*PS204 + C_P(P,2,7)*PS201 + C_P(P,3,7)*PS203 + C_P(P,5,7) - C_P(P,7,13)*PS193 + C_P(P,7,14)*PS75 + C_P(P,7,15)*PS190 + dt*(-C_P(P,0,4)*PS202 - C_P(P,1,4)*PS204 + C_P(P,2,4)*PS201 + C_P(P,3,4)*PS203 - C_P(P,4,13)*PS193 + C_P(P,4,14)*PS75 + C_P(P,4,15)*PS190 + C_P(P,4,5));
nextP_(7,8) = C_P(P,0,7)*PS216 + C_P(P,1,7)*PS217 - C_P(P,2,7)*PS214 + C_P(P,3,7)*PS215 + C_P(P,6,7) + C_P(P,7,13)*PS199 - C_P(P,7,14)*PS197 + C_P(P,7,15)*PS87 + dt*(C_P(P,0,4)*PS216 + C_P(P,1,4)*PS217 - C_P(P,2,4)*PS214 + C_P(P,3,4)*PS215 + C_P(P,4,13)*PS199 - C_P(P,4,14)*PS197 + C_P(P,4,15)*PS87 + C_P(P,4,6));
nextP_(8,8) = C_P(P,4,7)*dt + C_P(P,7,7) + dt*(C_P(P,4,4)*dt + C_P(P,4,7));

nextP_(1,9) = C_P(P,0,8) - C_P(P,1,8)*PS11 - C_P(P,2,8)*PS12 - C_P(P,3,8)*PS13 + C_P(P,8,10)*PS6 + C_P(P,8,11)*PS7 + C_P(P,8,12)*PS9 + PS86*dt;
nextP_(2,9) = C_P(P,0,8)*PS11 + C_P(P,1,8) + C_P(P,2,8)*PS13 - C_P(P,3,8)*PS12 - C_P(P,8,10)*PS34 + C_P(P,8,11)*PS9 - C_P(P,8,12)*PS7 + PS124*dt;
nextP_(3,9) = C_P(P,0,8)*PS12 - C_P(P,1,8)*PS13 + C_P(P,2,8) + C_P(P,3,8)*PS11 - C_P(P,8,10)*PS9 - C_P(P,8,11)*PS34 + C_P(P,8,12)*PS6 + PS149*dt;
nextP_(4,9) = C_P(P,0,8)*PS13 + C_P(P,1,8)*PS12 - C_P(P,2,8)*PS11 + C_P(P,3,8) + C_P(P,8,10)*PS7 - C_P(P,8,11)*PS6 - C_P(P,8,12)*PS34 + PS169*dt;
nextP_(5,9) = C_P(P,0,8)*PS174 + C_P(P,1,8)*PS173 + C_P(P,2,8)*PS175 - C_P(P,3,8)*PS176 + C_P(P,4,8) + C_P(P,8,13)*PS43 + C_P(P,8,14)*PS172 - C_P(P,8,15)*PS171 + PS196*dt;
nextP_(6,9) = -C_P(P,0,8)*PS202 - C_P(P,1,8)*PS204 + C_P(P,2,8)*PS201 + C_P(P,3,8)*PS203 + C_P(P,5,8) - C_P(P,8,13)*PS193 + C_P(P,8,14)*PS75 + C_P(P,8,15)*PS190 + PS213*dt;
nextP_(7,9) = C_P(P,0,8)*PS216 + C_P(P,1,8)*PS217 - C_P(P,2,8)*PS214 + C_P(P,3,8)*PS215 + C_P(P,6,8) + C_P(P,8,13)*PS199 - C_P(P,8,14)*PS197 + C_P(P,8,15)*PS87 + dt*(C_P(P,0,5)*PS216 + C_P(P,1,5)*PS217 - C_P(P,2,5)*PS214 + C_P(P,3,5)*PS215 + C_P(P,5,13)*PS199 - C_P(P,5,14)*PS197 + C_P(P,5,15)*PS87 + C_P(P,5,6));
nextP_(8,9) = C_P(P,4,8)*dt + C_P(P,7,8) + dt*(C_P(P,4,5)*dt + C_P(P,5,7));
nextP_(9,9) = C_P(P,5,8)*dt + C_P(P,8,8) + dt*(C_P(P,5,5)*dt + C_P(P,5,8));

nextP_(1,10) = C_P(P,0,9) - C_P(P,1,9)*PS11 - C_P(P,2,9)*PS12 - C_P(P,3,9)*PS13 + C_P(P,9,10)*PS6 + C_P(P,9,11)*PS7 + C_P(P,9,12)*PS9 + PS94*dt;
nextP_(2,10) = C_P(P,0,9)*PS11 + C_P(P,1,9) + C_P(P,2,9)*PS13 - C_P(P,3,9)*PS12 - C_P(P,9,10)*PS34 + C_P(P,9,11)*PS9 - C_P(P,9,12)*PS7 + PS125*dt;
nextP_(3,10) = C_P(P,0,9)*PS12 - C_P(P,1,9)*PS13 + C_P(P,2,9) + C_P(P,3,9)*PS11 - C_P(P,9,10)*PS9 - C_P(P,9,11)*PS34 + C_P(P,9,12)*PS6 + PS150*dt;
nextP_(4,10) = C_P(P,0,9)*PS13 + C_P(P,1,9)*PS12 - C_P(P,2,9)*PS11 + C_P(P,3,9) + C_P(P,9,10)*PS7 - C_P(P,9,11)*PS6 - C_P(P,9,12)*PS34 + PS170*dt;
nextP_(5,10) = C_P(P,0,9)*PS174 + C_P(P,1,9)*PS173 + C_P(P,2,9)*PS175 - C_P(P,3,9)*PS176 + C_P(P,4,9) + C_P(P,9,13)*PS43 + C_P(P,9,14)*PS172 - C_P(P,9,15)*PS171 + PS200*dt;
nextP_(6,10) = -C_P(P,0,9)*PS202 - C_P(P,1,9)*PS204 + C_P(P,2,9)*PS201 + C_P(P,3,9)*PS203 + C_P(P,5,9) - C_P(P,9,13)*PS193 + C_P(P,9,14)*PS75 + C_P(P,9,15)*PS190 + PS218*dt;
nextP_(7,10) = C_P(P,0,9)*PS216 + C_P(P,1,9)*PS217 - C_P(P,2,9)*PS214 + C_P(P,3,9)*PS215 + C_P(P,6,9) + C_P(P,9,13)*PS199 - C_P(P,9,14)*PS197 + C_P(P,9,15)*PS87 + PS222*dt;
nextP_(8,10) = C_P(P,4,9)*dt + C_P(P,7,9) + dt*(C_P(P,4,6)*dt + C_P(P,6,7));
nextP_(9,10) = C_P(P,5,9)*dt + C_P(P,8,9) + dt*(C_P(P,5,6)*dt + C_P(P,6,8));
nextP_(10,10) = C_P(P,6,9)*dt + C_P(P,9,9) + dt*(C_P(P,6,6)*dt + C_P(P,6,9));

nextP_(1,11) = PS14;
nextP_(2,11) = PS105;
nextP_(3,11) = PS133;
nextP_(4,11) = PS151;
nextP_(5,11) = C_P(P,0,10)*PS174 + C_P(P,1,10)*PS173 + C_P(P,10,13)*PS43 + C_P(P,10,14)*PS172 - C_P(P,10,15)*PS171 + C_P(P,2,10)*PS175 - C_P(P,3,10)*PS176 + C_P(P,4,10);
nextP_(6,11) = -C_P(P,0,10)*PS202 - C_P(P,1,10)*PS204 - C_P(P,10,13)*PS193 + C_P(P,10,14)*PS75 + C_P(P,10,15)*PS190 + C_P(P,2,10)*PS201 + C_P(P,3,10)*PS203 + C_P(P,5,10);
nextP_(7,11) = C_P(P,0,10)*PS216 + C_P(P,1,10)*PS217 + C_P(P,10,13)*PS199 - C_P(P,10,14)*PS197 + C_P(P,10,15)*PS87 - C_P(P,2,10)*PS214 + C_P(P,3,10)*PS215 + C_P(P,6,10);
nextP_(8,11) = C_P(P,4,10)*dt + C_P(P,7,10);
nextP_(9,11) = C_P(P,5,10)*dt + C_P(P,8,10);
nextP_(10,11) = C_P(P,6,10)*dt + C_P(P,9,10);
nextP_(11,11) = C_P(P,10,10);

nextP_(1,12) = PS17;
nextP_(2,12) = PS97;
nextP_(3,12) = PS132;
nextP_(4,12) = PS155;
nextP_(5,12) = C_P(P,0,11)*PS174 + C_P(P,1,11)*PS173 + C_P(P,11,13)*PS43 + C_P(P,11,14)*PS172 - C_P(P,11,15)*PS171 + C_P(P,2,11)*PS175 - C_P(P,3,11)*PS176 + C_P(P,4,11);
nextP_(6,12) = -C_P(P,0,11)*PS202 - C_P(P,1,11)*PS204 - C_P(P,11,13)*PS193 + C_P(P,11,14)*PS75 + C_P(P,11,15)*PS190 + C_P(P,2,11)*PS201 + C_P(P,3,11)*PS203 + C_P(P,5,11);
nextP_(7,12) = C_P(P,0,11)*PS216 + C_P(P,1,11)*PS217 + C_P(P,11,13)*PS199 - C_P(P,11,14)*PS197 + C_P(P,11,15)*PS87 - C_P(P,2,11)*PS214 + C_P(P,3,11)*PS215 + C_P(P,6,11);
nextP_(8,12) = C_P(P,4,11)*dt + C_P(P,7,11);
nextP_(9,12) = C_P(P,5,11)*dt + C_P(P,8,11);
nextP_(10,12) = C_P(P,6,11)*dt + C_P(P,9,11);
nextP_(11,12) = C_P(P,10,11);
nextP_(12,12) = C_P(P,11,11);

nextP_(1,13) = PS20;
nextP_(2,13) = PS107;
nextP_(3,13) = PS127;
nextP_(4,13) = PS154;
nextP_(5,13) = C_P(P,0,12)*PS174 + C_P(P,1,12)*PS173 + C_P(P,12,13)*PS43 + C_P(P,12,14)*PS172 - C_P(P,12,15)*PS171 + C_P(P,2,12)*PS175 - C_P(P,3,12)*PS176 + C_P(P,4,12);
nextP_(6,13) = -C_P(P,0,12)*PS202 - C_P(P,1,12)*PS204 - C_P(P,12,13)*PS193 + C_P(P,12,14)*PS75 + C_P(P,12,15)*PS190 + C_P(P,2,12)*PS201 + C_P(P,3,12)*PS203 + C_P(P,5,12);
nextP_(7,13) = C_P(P,0,12)*PS216 + C_P(P,1,12)*PS217 + C_P(P,12,13)*PS199 - C_P(P,12,14)*PS197 + C_P(P,12,15)*PS87 - C_P(P,2,12)*PS214 + C_P(P,3,12)*PS215 + C_P(P,6,12);
nextP_(8,13) = C_P(P,4,12)*dt + C_P(P,7,12);
nextP_(9,13) = C_P(P,5,12)*dt + C_P(P,8,12);
nextP_(10,13) = C_P(P,6,12)*dt + C_P(P,9,12);
nextP_(11,13) = C_P(P,10,12);
nextP_(12,13) = C_P(P,11,12);
nextP_(13,13) = C_P(P,12,12);
% add process noise that is not from the IMU
% process noise contribution for delta velocity states can be very small compared to
% the variances, therefore use algorithm to minimise numerical error
for i = 11:13
    nextP_(i,i) = kahanSummation(nextP_(i,i),process_noise(i),0);
end

%% calculate variances and upper diagonal covariances for IMU X AXIS DELTA VELOCITY BIAS state
if ~accel_bias_inhibit(1) == 1
    nextP_(1,14) = PS44;
    nextP_(2,14) = PS113;
    nextP_(3,14) = PS138;
    nextP_(4,14) = PS158;
    nextP_(5,14) = PS177;
    nextP_(6,14) = PS206;
    nextP_(7,14) = PS221;
    nextP_(8,14) = C_P(P,4,13)*dt + C_P(P,7,13);
    nextP_(9,14) = C_P(P,5,13)*dt + C_P(P,8,13);
    nextP_(10,14) = C_P(P,6,13)*dt + C_P(P,9,13);
    nextP_(11,14) = C_P(P,10,13);
    nextP_(12,14) = C_P(P,11,13);
    nextP_(13,14) = C_P(P,12,13);
    nextP_(14,14) = C_P(P,13,13);
    % add process noise that is not from the IMU
    % process noise contribution for delta velocity states can be very small compared to
    % the variances, therefore use algorithm to minimise numerical error
    nextP_(14,14) = kahanSummation(nextP_(14,14),process_noise(14),0);
end
%% calculate variances and upper diagonal covariances for IMU Y AXIS DELTA VELOCITY BIAS state
if ~accel_bias_inhibit(2) == 1
    nextP_(1,15) = PS57;
    nextP_(2,15) = PS117;
    nextP_(3,15) = PS142;
    nextP_(4,15) = PS162;
    nextP_(5,15) = PS180;
    nextP_(6,15) = PS205;
    nextP_(7,15) = PS220;
    nextP_(8,15) = C_P(P,4,14)*dt + C_P(P,7,14);
    nextP_(9,15) = C_P(P,5,14)*dt + C_P(P,8,14);
    nextP_(10,15) = C_P(P,6,14)*dt + C_P(P,9,14);
    nextP_(11,15) = C_P(P,10,14);
    nextP_(12,15) = C_P(P,11,14);
    nextP_(13,15) = C_P(P,12,14);
    nextP_(14,15) = C_P(P,13,14);
    nextP_(15,15) = C_P(P,14,14);
    % add process noise that is not from the IMU
    % process noise contribution for delta velocity states can be very small compared to
    % the variances, therefore use algorithm to minimise numerical error
    nextP_(15,15) = kahanSummation(nextP_(15,15),process_noise(15),0);
end
%% calculate variances and upper diagonal covariances for IMU Z AXIS DELTA VELOCITY BIAS state
if ~accel_bias_inhibit(3) == 1
    nextP_(1,16) = PS46;
    nextP_(2,16) = PS114;
    nextP_(3,16) = PS139;
    nextP_(4,16) = PS159;
    nextP_(5,16) = PS178;
    nextP_(6,16) = PS209;
    nextP_(7,16) = PS219;
    nextP_(8,16) = C_P(P,4,15)*dt + C_P(P,7,15);
    nextP_(9,16) = C_P(P,5,15)*dt + C_P(P,8,15);
    nextP_(10,16) = C_P(P,6,15)*dt + C_P(P,9,15);
    nextP_(11,16) = C_P(P,10,15);
    nextP_(12,16) = C_P(P,11,15);
    nextP_(13,16) = C_P(P,12,15);
    nextP_(14,16) = C_P(P,13,15);
    nextP_(15,16) = C_P(P,14,15);
    nextP_(16,16) = C_P(P,15,15);
    % add process noise that is not from the IMU
    % process noise contribution for delta velocity states can be very small compared to
    % the variances, therefore use algorithm to minimise numerical error
    nextP_(16,16) = kahanSummation(nextP_(16,16),process_noise(16),0);
end
%% Don't do covariance prediction on MAGNETIC FIELD states unless we are using 3-axis fusion
if control_status_flags.mag_3D == 1
    % calculate variances and upper diagonal covariances for earth and body magnetic field states
    nextP_(1,17) = C_P(P,0,16) - C_P(P,1,16)*PS11 + C_P(P,10,16)*PS6 + C_P(P,11,16)*PS7 + C_P(P,12,16)*PS9 - C_P(P,2,16)*PS12 - C_P(P,3,16)*PS13;
    nextP_(2,17) = C_P(P,0,16)*PS11 + C_P(P,1,16) - C_P(P,10,16)*PS34 + C_P(P,11,16)*PS9 - C_P(P,12,16)*PS7 + C_P(P,2,16)*PS13 - C_P(P,3,16)*PS12;
    nextP_(3,17) = C_P(P,0,16)*PS12 - C_P(P,1,16)*PS13 - C_P(P,10,16)*PS9 - C_P(P,11,16)*PS34 + C_P(P,12,16)*PS6 + C_P(P,2,16) + C_P(P,3,16)*PS11;
    nextP_(4,17) = C_P(P,0,16)*PS13 + C_P(P,1,16)*PS12 + C_P(P,10,16)*PS7 - C_P(P,11,16)*PS6 - C_P(P,12,16)*PS34 - C_P(P,2,16)*PS11 + C_P(P,3,16);
    nextP_(5,17) = C_P(P,0,16)*PS174 + C_P(P,1,16)*PS173 + C_P(P,13,16)*PS43 + C_P(P,14,16)*PS172 - C_P(P,15,16)*PS171 + C_P(P,2,16)*PS175 - C_P(P,3,16)*PS176 + C_P(P,4,16);
    nextP_(6,17) = -C_P(P,0,16)*PS202 - C_P(P,1,16)*PS204 - C_P(P,13,16)*PS193 + C_P(P,14,16)*PS75 + C_P(P,15,16)*PS190 + C_P(P,2,16)*PS201 + C_P(P,3,16)*PS203 + C_P(P,5,16);
    nextP_(7,17) = C_P(P,0,16)*PS216 + C_P(P,1,16)*PS217 + C_P(P,13,16)*PS199 - C_P(P,14,16)*PS197 + C_P(P,15,16)*PS87 - C_P(P,2,16)*PS214 + C_P(P,3,16)*PS215 + C_P(P,6,16);
    nextP_(8,17) = C_P(P,4,16)*dt + C_P(P,7,16);
    nextP_(9,17) = C_P(P,5,16)*dt + C_P(P,8,16);
    nextP_(10,17) = C_P(P,6,16)*dt + C_P(P,9,16);
    nextP_(11,17) = C_P(P,10,16);
    nextP_(12,17) = C_P(P,11,16);
    nextP_(13,17) = C_P(P,12,16);
    nextP_(14,17) = C_P(P,13,16);
    nextP_(15,17) = C_P(P,14,16);
    nextP_(16,17) = C_P(P,15,16);
    nextP_(17,17) = C_P(P,16,16);
    
    nextP_(1,18) = C_P(P,0,17) - C_P(P,1,17)*PS11 + C_P(P,10,17)*PS6 + C_P(P,11,17)*PS7 + C_P(P,12,17)*PS9 - C_P(P,2,17)*PS12 - C_P(P,3,17)*PS13;
    nextP_(2,18) = C_P(P,0,17)*PS11 + C_P(P,1,17) - C_P(P,10,17)*PS34 + C_P(P,11,17)*PS9 - C_P(P,12,17)*PS7 + C_P(P,2,17)*PS13 - C_P(P,3,17)*PS12;
    nextP_(3,18) = C_P(P,0,17)*PS12 - C_P(P,1,17)*PS13 - C_P(P,10,17)*PS9 - C_P(P,11,17)*PS34 + C_P(P,12,17)*PS6 + C_P(P,2,17) + C_P(P,3,17)*PS11;
    nextP_(4,18) = C_P(P,0,17)*PS13 + C_P(P,1,17)*PS12 + C_P(P,10,17)*PS7 - C_P(P,11,17)*PS6 - C_P(P,12,17)*PS34 - C_P(P,2,17)*PS11 + C_P(P,3,17);
    nextP_(5,18) = C_P(P,0,17)*PS174 + C_P(P,1,17)*PS173 + C_P(P,13,17)*PS43 + C_P(P,14,17)*PS172 - C_P(P,15,17)*PS171 + C_P(P,2,17)*PS175 - C_P(P,3,17)*PS176 + C_P(P,4,17);
    nextP_(6,18) = -C_P(P,0,17)*PS202 - C_P(P,1,17)*PS204 - C_P(P,13,17)*PS193 + C_P(P,14,17)*PS75 + C_P(P,15,17)*PS190 + C_P(P,2,17)*PS201 + C_P(P,3,17)*PS203 + C_P(P,5,17);
    nextP_(7,18) = C_P(P,0,17)*PS216 + C_P(P,1,17)*PS217 + C_P(P,13,17)*PS199 - C_P(P,14,17)*PS197 + C_P(P,15,17)*PS87 - C_P(P,2,17)*PS214 + C_P(P,3,17)*PS215 + C_P(P,6,17);
    nextP_(8,18) = C_P(P,4,17)*dt + C_P(P,7,17);
    nextP_(9,18) = C_P(P,5,17)*dt + C_P(P,8,17);
    nextP_(10,18) = C_P(P,6,17)*dt + C_P(P,9,17);
    nextP_(11,18) = C_P(P,10,17);
    nextP_(12,18) = C_P(P,11,17);
    nextP_(13,18) = C_P(P,12,17);
    nextP_(14,18) = C_P(P,13,17);
    nextP_(15,18) = C_P(P,14,17);
    nextP_(16,18) = C_P(P,15,17);
    nextP_(17,18) = C_P(P,16,17);
    nextP_(18,18) = C_P(P,17,17);
    
    nextP_(1,19) = C_P(P,0,18) - C_P(P,1,18)*PS11 + C_P(P,10,18)*PS6 + C_P(P,11,18)*PS7 + C_P(P,12,18)*PS9 - C_P(P,2,18)*PS12 - C_P(P,3,18)*PS13;
    nextP_(2,19) = C_P(P,0,18)*PS11 + C_P(P,1,18) - C_P(P,10,18)*PS34 + C_P(P,11,18)*PS9 - C_P(P,12,18)*PS7 + C_P(P,2,18)*PS13 - C_P(P,3,18)*PS12;
    nextP_(3,19) = C_P(P,0,18)*PS12 - C_P(P,1,18)*PS13 - C_P(P,10,18)*PS9 - C_P(P,11,18)*PS34 + C_P(P,12,18)*PS6 + C_P(P,2,18) + C_P(P,3,18)*PS11;
    nextP_(4,19) = C_P(P,0,18)*PS13 + C_P(P,1,18)*PS12 + C_P(P,10,18)*PS7 - C_P(P,11,18)*PS6 - C_P(P,12,18)*PS34 - C_P(P,2,18)*PS11 + C_P(P,3,18);
    nextP_(5,19) = C_P(P,0,18)*PS174 + C_P(P,1,18)*PS173 + C_P(P,13,18)*PS43 + C_P(P,14,18)*PS172 - C_P(P,15,18)*PS171 + C_P(P,2,18)*PS175 - C_P(P,3,18)*PS176 + C_P(P,4,18);
    nextP_(6,19) = -C_P(P,0,18)*PS202 - C_P(P,1,18)*PS204 - C_P(P,13,18)*PS193 + C_P(P,14,18)*PS75 + C_P(P,15,18)*PS190 + C_P(P,2,18)*PS201 + C_P(P,3,18)*PS203 + C_P(P,5,18);
    nextP_(7,19) = C_P(P,0,18)*PS216 + C_P(P,1,18)*PS217 + C_P(P,13,18)*PS199 - C_P(P,14,18)*PS197 + C_P(P,15,18)*PS87 - C_P(P,2,18)*PS214 + C_P(P,3,18)*PS215 + C_P(P,6,18);
    nextP_(8,19) = C_P(P,4,18)*dt + C_P(P,7,18);
    nextP_(9,19) = C_P(P,5,18)*dt + C_P(P,8,18);
    nextP_(10,19) = C_P(P,6,18)*dt + C_P(P,9,18);
    nextP_(11,19) = C_P(P,10,18);
    nextP_(12,19) = C_P(P,11,18);
    nextP_(13,19) = C_P(P,12,18);
    nextP_(14,19) = C_P(P,13,18);
    nextP_(15,19) = C_P(P,14,18);
    nextP_(16,19) = C_P(P,15,18);
    nextP_(17,19) = C_P(P,16,18);
    nextP_(18,19) = C_P(P,17,18);
    nextP_(19,19) = C_P(P,18,18);
    
    nextP_(1,20) = C_P(P,0,19) - C_P(P,1,19)*PS11 + C_P(P,10,19)*PS6 + C_P(P,11,19)*PS7 + C_P(P,12,19)*PS9 - C_P(P,2,19)*PS12 - C_P(P,3,19)*PS13;
    nextP_(2,20) = C_P(P,0,19)*PS11 + C_P(P,1,19) - C_P(P,10,19)*PS34 + C_P(P,11,19)*PS9 - C_P(P,12,19)*PS7 + C_P(P,2,19)*PS13 - C_P(P,3,19)*PS12;
    nextP_(3,20) = C_P(P,0,19)*PS12 - C_P(P,1,19)*PS13 - C_P(P,10,19)*PS9 - C_P(P,11,19)*PS34 + C_P(P,12,19)*PS6 + C_P(P,2,19) + C_P(P,3,19)*PS11;
    nextP_(4,20) = C_P(P,0,19)*PS13 + C_P(P,1,19)*PS12 + C_P(P,10,19)*PS7 - C_P(P,11,19)*PS6 - C_P(P,12,19)*PS34 - C_P(P,2,19)*PS11 + C_P(P,3,19);
    nextP_(5,20) = C_P(P,0,19)*PS174 + C_P(P,1,19)*PS173 + C_P(P,13,19)*PS43 + C_P(P,14,19)*PS172 - C_P(P,15,19)*PS171 + C_P(P,2,19)*PS175 - C_P(P,3,19)*PS176 + C_P(P,4,19);
    nextP_(6,20) = -C_P(P,0,19)*PS202 - C_P(P,1,19)*PS204 - C_P(P,13,19)*PS193 + C_P(P,14,19)*PS75 + C_P(P,15,19)*PS190 + C_P(P,2,19)*PS201 + C_P(P,3,19)*PS203 + C_P(P,5,19);
    nextP_(1,20) = C_P(P,0,19)*PS216 + C_P(P,1,19)*PS217 + C_P(P,13,19)*PS199 - C_P(P,14,19)*PS197 + C_P(P,15,19)*PS87 - C_P(P,2,19)*PS214 + C_P(P,3,19)*PS215 + C_P(P,6,19);
    nextP_(8,20) = C_P(P,4,19)*dt + C_P(P,7,19);
    nextP_(9,20) = C_P(P,5,19)*dt + C_P(P,8,19);
    nextP_(10,20) = C_P(P,6,19)*dt + C_P(P,9,19);
    nextP_(11,20) = C_P(P,10,19);
    nextP_(12,20) = C_P(P,11,19);
    nextP_(13,20) = C_P(P,12,19);
    nextP_(14,20) = C_P(P,13,19);
    nextP_(18,20) = C_P(P,14,19);
    nextP_(16,20) = C_P(P,15,19);
    nextP_(17,20) = C_P(P,16,19);
    nextP_(18,20) = C_P(P,17,19);
    nextP_(19,20) = C_P(P,18,19);
    nextP_(20,20) = C_P(P,19,19);
    
    nextP_(1,21) = C_P(P,0,20) - C_P(P,1,20)*PS11 + C_P(P,10,20)*PS6 + C_P(P,11,20)*PS7 + C_P(P,12,20)*PS9 - C_P(P,2,20)*PS12 - C_P(P,3,20)*PS13;
    nextP_(2,21) = C_P(P,0,20)*PS11 + C_P(P,1,20) - C_P(P,10,20)*PS34 + C_P(P,11,20)*PS9 - C_P(P,12,20)*PS7 + C_P(P,2,20)*PS13 - C_P(P,3,20)*PS12;
    nextP_(3,21) = C_P(P,0,20)*PS12 - C_P(P,1,20)*PS13 - C_P(P,10,20)*PS9 - C_P(P,11,20)*PS34 + C_P(P,12,20)*PS6 + C_P(P,2,20) + C_P(P,3,20)*PS11;
    nextP_(4,21) = C_P(P,0,20)*PS13 + C_P(P,1,20)*PS12 + C_P(P,10,20)*PS7 - C_P(P,11,20)*PS6 - C_P(P,12,20)*PS34 - C_P(P,2,20)*PS11 + C_P(P,3,20);
    nextP_(5,21) = C_P(P,0,20)*PS174 + C_P(P,1,20)*PS173 + C_P(P,13,20)*PS43 + C_P(P,14,20)*PS172 - C_P(P,15,20)*PS171 + C_P(P,2,20)*PS175 - C_P(P,3,20)*PS176 + C_P(P,4,20);
    nextP_(6,21) = -C_P(P,0,20)*PS202 - C_P(P,1,20)*PS204 - C_P(P,13,20)*PS193 + C_P(P,14,20)*PS75 + C_P(P,15,20)*PS190 + C_P(P,2,20)*PS201 + C_P(P,3,20)*PS203 + C_P(P,5,20);
    nextP_(7,21) = C_P(P,0,20)*PS216 + C_P(P,1,20)*PS217 + C_P(P,13,20)*PS199 - C_P(P,14,20)*PS197 + C_P(P,15,20)*PS87 - C_P(P,2,20)*PS214 + C_P(P,3,20)*PS215 + C_P(P,6,20);
    nextP_(8,21) = C_P(P,4,20)*dt + C_P(P,7,20);
    nextP_(9,21) = C_P(P,5,20)*dt + C_P(P,8,20);
    nextP_(10,21) = C_P(P,6,20)*dt + C_P(P,9,20);
    nextP_(11,21) = C_P(P,10,20);
    nextP_(15,21) = C_P(P,11,20);
    nextP_(13,21) = C_P(P,12,20);
    nextP_(14,21) = C_P(P,13,20);
    nextP_(15,21) = C_P(P,14,20);
    nextP_(16,21) = C_P(P,15,20);
    nextP_(17,21) = C_P(P,16,20);
    nextP_(18,21) = C_P(P,17,20);
    nextP_(19,21) = C_P(P,18,20);
    nextP_(20,21) = C_P(P,19,20);
    nextP_(21,21) = C_P(P,20,20);
    
    nextP_(1,22) = C_P(P,0,21) - C_P(P,1,21)*PS11 + C_P(P,10,21)*PS6 + C_P(P,11,21)*PS7 + C_P(P,12,21)*PS9 - C_P(P,2,21)*PS12 - C_P(P,3,21)*PS13;
    nextP_(2,22) = C_P(P,0,21)*PS11 + C_P(P,1,21) - C_P(P,10,21)*PS34 + C_P(P,11,21)*PS9 - C_P(P,12,21)*PS7 + C_P(P,2,21)*PS13 - C_P(P,3,21)*PS12;
    nextP_(3,22) = C_P(P,0,21)*PS12 - C_P(P,1,21)*PS13 - C_P(P,10,21)*PS9 - C_P(P,11,21)*PS34 + C_P(P,12,21)*PS6 + C_P(P,2,21) + C_P(P,3,21)*PS11;
    nextP_(4,22) = C_P(P,0,21)*PS13 + C_P(P,1,21)*PS12 + C_P(P,10,21)*PS7 - C_P(P,11,21)*PS6 - C_P(P,12,21)*PS34 - C_P(P,2,21)*PS11 + C_P(P,3,21);
    nextP_(5,22) = C_P(P,0,21)*PS174 + C_P(P,1,21)*PS173 + C_P(P,13,21)*PS43 + C_P(P,14,21)*PS172 - C_P(P,15,21)*PS171 + C_P(P,2,21)*PS175 - C_P(P,3,21)*PS176 + C_P(P,4,21);
    nextP_(6,22) = -C_P(P,0,21)*PS202 - C_P(P,1,21)*PS204 - C_P(P,13,21)*PS193 + C_P(P,14,21)*PS75 + C_P(P,15,21)*PS190 + C_P(P,2,21)*PS201 + C_P(P,3,21)*PS203 + C_P(P,5,21);
    nextP_(7,22) = C_P(P,0,21)*PS216 + C_P(P,1,21)*PS217 + C_P(P,13,21)*PS199 - C_P(P,14,21)*PS197 + C_P(P,15,21)*PS87 - C_P(P,2,21)*PS214 + C_P(P,3,21)*PS215 + C_P(P,6,21);
    nextP_(8,22) = C_P(P,4,21)*dt + C_P(P,7,21);
    nextP_(9,22) = C_P(P,5,21)*dt + C_P(P,8,21);
    nextP_(10,22) = C_P(P,6,21)*dt + C_P(P,9,21);
    nextP_(11,22) = C_P(P,10,21);
    nextP_(12,22) = C_P(P,11,21);
    nextP_(13,22) = C_P(P,12,21);
    nextP_(14,22) = C_P(P,13,21);
    nextP_(15,22) = C_P(P,14,21);
    nextP_(16,22) = C_P(P,15,21);
    nextP_(17,22) = C_P(P,16,21);
    nextP_(18,22) = C_P(P,17,21);
    nextP_(19,22) = C_P(P,18,21);
    nextP_(20,22) = C_P(P,19,21);
    nextP_(21,22) = C_P(P,20,21);
    nextP_(22,22) = C_P(P,21,21);
    % add process noise that is not from the IMU
    for i=14:22
        nextP_(i, i) = nextP_(i, i)+process_noise(i);
    end
end

%% Don't do covariance prediction on wind states unless we are using them
if control_status_flags.wind == 1
    % calculate variances and upper diagonal covariances for wind states
    nextP_(1,23) = C_P(P,0,22) - C_P(P,1,22)*PS11 + C_P(P,10,22)*PS6 + C_P(P,11,22)*PS7 + C_P(P,12,22)*PS9 - C_P(P,2,22)*PS12 - C_P(P,3,22)*PS13;
    nextP_(2,23) = C_P(P,0,22)*PS11 + C_P(P,1,22) - C_P(P,10,22)*PS34 + C_P(P,11,22)*PS9 - C_P(P,12,22)*PS7 + C_P(P,2,22)*PS13 - C_P(P,3,22)*PS12;
    nextP_(3,23) = C_P(P,0,22)*PS12 - C_P(P,1,22)*PS13 - C_P(P,10,22)*PS9 - C_P(P,11,22)*PS34 + C_P(P,12,22)*PS6 + C_P(P,2,22) + C_P(P,3,22)*PS11;
    nextP_(4,23) = C_P(P,0,22)*PS13 + C_P(P,1,22)*PS12 + C_P(P,10,22)*PS7 - C_P(P,11,22)*PS6 - C_P(P,12,22)*PS34 - C_P(P,2,22)*PS11 + C_P(P,3,22);
    nextP_(5,23) = C_P(P,0,22)*PS174 + C_P(P,1,22)*PS173 + C_P(P,13,22)*PS43 + C_P(P,14,22)*PS172 - C_P(P,15,22)*PS171 + C_P(P,2,22)*PS175 - C_P(P,3,22)*PS176 + C_P(P,4,22);
    nextP_(6,23) = -C_P(P,0,22)*PS202 - C_P(P,1,22)*PS204 - C_P(P,13,22)*PS193 + C_P(P,14,22)*PS75 + C_P(P,15,22)*PS190 + C_P(P,2,22)*PS201 + C_P(P,3,22)*PS203 + C_P(P,5,22);
    nextP_(7,23) = C_P(P,0,22)*PS216 + C_P(P,1,22)*PS217 + C_P(P,13,22)*PS199 - C_P(P,14,22)*PS197 + C_P(P,15,22)*PS87 - C_P(P,2,22)*PS214 + C_P(P,3,22)*PS215 + C_P(P,6,22);
    nextP_(8,23) = C_P(P,4,22)*dt + C_P(P,7,22);
    nextP_(9,23) = C_P(P,5,22)*dt + C_P(P,8,22);
    nextP_(10,23) = C_P(P,6,22)*dt + C_P(P,9,22);
    nextP_(11,23) = C_P(P,10,22);
    nextP_(12,23) = C_P(P,11,22);
    nextP_(13,23) = C_P(P,12,22);
    nextP_(14,23) = C_P(P,13,22);
    nextP_(15,23) = C_P(P,14,22);
    nextP_(16,23) = C_P(P,15,22);
    nextP_(17,23) = C_P(P,16,22);
    nextP_(18,23) = C_P(P,17,22);
    nextP_(19,23) = C_P(P,18,22);
    nextP_(20,23) = C_P(P,19,22);
    nextP_(21,23) = C_P(P,20,22);
    nextP_(22,23) = C_P(P,21,22);
    nextP_(23,23) = C_P(P,22,22);
    nextP_(1,24) = C_P(P,0,23) - C_P(P,1,23)*PS11 + C_P(P,10,23)*PS6 + C_P(P,11,23)*PS7 + C_P(P,12,23)*PS9 - C_P(P,2,23)*PS12 - C_P(P,3,23)*PS13;
    nextP_(2,24) = C_P(P,0,23)*PS11 + C_P(P,1,23) - C_P(P,10,23)*PS34 + C_P(P,11,23)*PS9 - C_P(P,12,23)*PS7 + C_P(P,2,23)*PS13 - C_P(P,3,23)*PS12;
    nextP_(3,24) = C_P(P,0,23)*PS12 - C_P(P,1,23)*PS13 - C_P(P,10,23)*PS9 - C_P(P,11,23)*PS34 + C_P(P,12,23)*PS6 + C_P(P,2,23) + C_P(P,3,23)*PS11;
    nextP_(4,24) = C_P(P,0,23)*PS13 + C_P(P,1,23)*PS12 + C_P(P,10,23)*PS7 - C_P(P,11,23)*PS6 - C_P(P,12,23)*PS34 - C_P(P,2,23)*PS11 + C_P(P,3,23);
    nextP_(5,24) = C_P(P,0,23)*PS174 + C_P(P,1,23)*PS173 + C_P(P,13,23)*PS43 + C_P(P,14,23)*PS172 - C_P(P,15,23)*PS171 + C_P(P,2,23)*PS175 - C_P(P,3,23)*PS176 + C_P(P,4,23);
    nextP_(6,24) = -C_P(P,0,23)*PS202 - C_P(P,1,23)*PS204 - C_P(P,13,23)*PS193 + C_P(P,14,23)*PS75 + C_P(P,15,23)*PS190 + C_P(P,2,23)*PS201 + C_P(P,3,23)*PS203 + C_P(P,5,23);
    nextP_(7,24) = C_P(P,0,23)*PS216 + C_P(P,1,23)*PS217 + C_P(P,13,23)*PS199 - C_P(P,14,23)*PS197 + C_P(P,15,23)*PS87 - C_P(P,2,23)*PS214 + C_P(P,3,23)*PS215 + C_P(P,6,23);
    nextP_(8,23) = C_P(P,4,23)*dt + C_P(P,7,23);
    nextP_(9,24) = C_P(P,5,23)*dt + C_P(P,8,23);
    nextP_(10,24) = C_P(P,6,23)*dt + C_P(P,9,23);
    nextP_(11,24) = C_P(P,10,23);
    nextP_(12,24) = C_P(P,11,23);
    nextP_(13,24) = C_P(P,12,23);
    nextP_(14,24) = C_P(P,13,23);
    nextP_(15,24) = C_P(P,14,23);
    nextP_(16,24) = C_P(P,15,23);
    nextP_(17,24) = C_P(P,16,23);
    nextP_(18,24) = C_P(P,17,23);
    nextP_(19,24) = C_P(P,18,23);
    nextP_(20,24) = C_P(P,19,23);
    nextP_(21,24) = C_P(P,20,23);
    nextP_(22,24) = C_P(P,21,23);
    nextP_(23,24) = C_P(P,22,23);
    nextP_(24,24) = C_P(P,23,23);
    % add process noise that is not from the IMU
    for i = 23:24
	    nextP_(i, i) = nextP_(i, i)+process_noise(i);
    end
end

%% covariance matrix is symmetrical, so copy upper half to lower half
for row = 2:24
    for column = 1:23
        P(column, row) = nextP_(column, row);
        P(row, column) = nextP_(column, row) ;
    end
end

%% copy variances (diagonals)
for i = 1:24
    P(i, i) = nextP_(i, i);
end
P = fixCovarianceErrors(P,1);

== matlab function AFCToolbox2023a/基础导航算法模型库/ECL EKF/Subsystem/Subsystem2/Predict States ==
  data: corrected_delta_ang output; corrected_delta_vel output; states input single; states output; delta_ang input; delta_vel input; dt input; latitude input
function [corrected_delta_ang,corrected_delta_vel,states]= PredictStates(...
    states,...   % previous state vector (4x1 quaternion, 3x1 velocity, 3x1 position, 3x1 delAng bias, 3x1 delVel bias)
    delta_ang,...% IMU delta angle measurements, 3x1 (rad)
    delta_vel,...% IMU delta velocity measurements 3x1 (m/s)
    dt,...       % accumulation time of the IMU measurement (sec)
    latitude)% WGS-84 latitude (rad)

persistent Tbn_prev;
if isempty(Tbn_prev)
    % Rotation from BODY coordinate system to NAVIGATION coordinate,B→N
    Tbn_prev = Quat2Tbn(states(1:4));
end
% acceleration due to gravity (m/s/s)
gravity = 9.80665;

%% Propagation of quaternion states
% apply imu bias corrections:                               Δθm-Δθb
corrected_delta_ang = delta_ang - states(11:13);
% Calculate earth rate NED(rad/s)
% ~ gps_chercks.cpp -> collect_gps(...) ~ ekf_heper.cpp -> calcEarthRateNED(...)
earth_rate_NED = [0.000072921 * cos(latitude);
                                          0.0;
                 -0.000072921 * sin(latitude)];
% Calculate earth delta angle spin vector:                  Δθearth=Tnb*Vearth_NED*Δt
delta_ang_earth_NED = earth_rate_NED*dt;
delta_ang_earth = transpose(Tbn_prev)*delta_ang_earth_NED;
% Subtract component of angular rate due to earth rotation: Δθtruth=Δθm-Δθb-Δθearth
% calculate the true angular increment
corrected_delta_ang = corrected_delta_ang - delta_ang_earth;

% Convert the rotation vector to its equivalent quaternion: M(Δqk)
M_delta_Quat = angToQuatMult(corrected_delta_ang);
% rotate the previous quaternion by the delta quaternion using a quaternion multiplication:qk*M(Δqk)
states(1:4) = M_delta_Quat*states(1:4);
states(1:4) = normQuat(states(1:4));

Tbn = Quat2Tbn(states(1:4));
Tbn_prev = Tbn;

%% Propagation of velocity:                                 vk+1=vk+RB→N*Δv+gN*Δt
% Calculate true delta velocity:                            Δv=(Δvm-Δvn)-Δvb
corrected_delta_vel = delta_vel - states(14:16);
% Calculate an earth frame(NED) delta velocity:             RB→N*Δv
corrected_delta_vel_ef = Tbn_prev*corrected_delta_vel;
% save the previous value of velocity so we can use trapzoidal integration
vel_last = states(5:7);
% calculate the increment in velocity using the current orientation:vk+1=vk+RN→B*Δv
states(5:7) = states(5:7) + corrected_delta_vel_ef;
% Consider gravity acceleration compensation:               gN*Δt
states(5:7) = states(5:7) + [0;0;gravity]*dt;

%% Propagation of position:                                 pk+1=pk+0.5*(vk+vk+1)*Δt                              
states(8:10) = states(8:10) + 0.5*(vel_last + states(5:7))*dt;

%% constrainStates
[states]  = ConstrainStates(states,dt);

== matlab function AFCToolbox2023a/基础导航算法模型库/ECL EKF/init_state/InitState_accel1/initAccel1 ==
  data: QGCinitflag input; init_vel output; GPSfixtype input; imu_data_del_vel input; init_GPSflag output
function [init_vel,init_GPSflag] = initAccel(QGCinitflag,GPSfixtype,imu_data_del_vel)
    persistent initGPSflag;
    persistent initVel;

    if isempty(initGPSflag)
        initGPSflag = 0;
    end
    if isempty(initVel)
        % 初始GPS未进入定位状态，给定值
        initVel = zeros(3,1);
 
    end
    if (initGPSflag == 0 && GPSfixtype >= 1) || (QGCinitflag == 1 && GPSfixtype >= 1)
        % 当GPS第一次初始化位置时，当GPSfixtype >=1 时，自动初始化一次位置，initGPSLLAflag置1
        % 或者是利用QGCinitflag地面站重新修正，不过需要满足GPSfixtype>=1的条件
        initVel = imu_data_del_vel;       
        initGPSflag = 1;
    end
    init_vel = initVel;
    init_GPSflag = initGPSflag;
end

== matlab function AFCToolbox2023a/SimuMoudle/Position-Control/Consistent formation control /一致性控制——F2/MATLAB Function3 ==
  data: r input; result output
function result = Faixy(r)
%UNTITLED 此处显示有关此函数的摘要


result=-1.8*(1-exp(-0.5*r))/(1+exp(-0.5*r));



end

== matlab function AFCToolbox2023a/基础导航算法模型库/ECL EKF/init_state/InitState_baro1/MATLAB Function ==
  data: pressure_pa input; altitude output
function altitude = PressureToAltitude(pressure_pa)
% VehicleAirData.cpp -> PressureToAltitude(...)
CONSTANTS_ABSOLUTE_NULL_CELSIUS = 273.15; % °C
CONSTANTS_AIR_GAS_CONST = 287.1; %J/(kg * K)
CONSTANTS_ONE_G = 9.80665;
% calculate altitude using the hypsometric equation
T1 = 15 - CONSTANTS_ABSOLUTE_NULL_CELSIUS; % temperature at base height in Kelvin
a = -6.5 / 1000; % temperature gradient in degrees per metre

% current pressure at MSL in kPa (QNH in hPa)
param_sens_baro_qnh.get = 1007;% Shenzhen's Baro
p1 = param_sens_baro_qnh.get() * 0.1;

% measured pressure in kPa
p = pressure_pa * 0.001;

% /*
%  * Solve:
%  *
%  *     /        -(aR / g)     \
%  *    | (p / p1)          . T1 | - T1
%  *     \                      /
%  * h = -------------------------------  + h1
%  *                   a
%  */
altitude = (((power((p / p1), (-(a * CONSTANTS_AIR_GAS_CONST) / CONSTANTS_ONE_G))) * T1) - T1) / a;
